simulink model "FMT_QuadPlantStep"  (R2026b)
settings: Solver=FixedStepDiscrete  StopTime=2  FixedStep=0.0005
undefined symbols (not defined in the file): PlantStepS
settings Model: DataDictionary=Flight_Parameters.sldd  Creator=26718  LastModifiedBy=26718

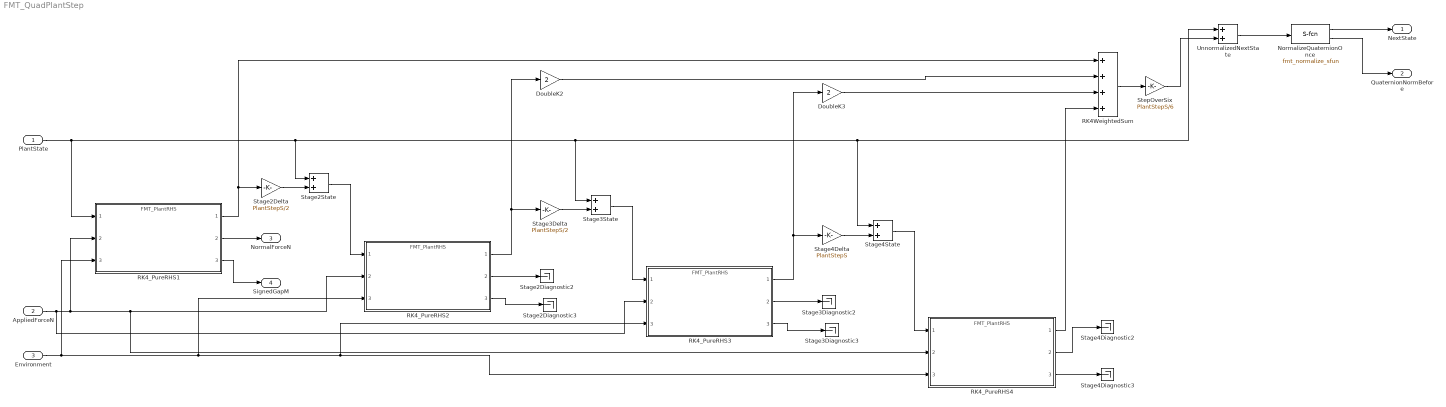
== system FMT_QuadPlantStep ==
  PlantState : Inport  OutDataTypeStr=double  PortDimensions=17
  AppliedForceN : Inport  Port=2  OutDataTypeStr=double  PortDimensions=4
  Environment : Inport  Port=3  OutDataTypeStr=double  PortDimensions=15
  DoubleK2 : Gain  Gain=2
  DoubleK3 : Gain  Gain=2
  NormalizeQuaternionOnce : S-Function  FunctionName=fmt_normalize_sfun  SFunctionDeploymentMode=off  EnableBusSupport=off
  RK4WeightedSum : Sum  Inputs=++++
  RK4_PureRHS{1..4} (4 alike) : ModelReference  ModelNameDialog=FMT_PlantRHS  SimulationMode=Normal  ModelReferenceVersion=1.1
  Stage2Delta : Gain  Gain=PlantStepS/2
  Stage2Diagnostic2 : Terminator
  Stage2Diagnostic3 : Terminator
  Stage2State : Sum
  Stage3Delta : Gain  Gain=PlantStepS/2
  Stage3Diagnostic2 : Terminator
  Stage3Diagnostic3 : Terminator
  Stage3State : Sum
  Stage4Delta : Gain  Gain=PlantStepS
  Stage4Diagnostic2 : Terminator
  Stage4Diagnostic3 : Terminator
  Stage4State : Sum
  StepOverSix : Gain  Gain=PlantStepS/6
  UnnormalizedNextState : Sum
  NextState : Outport
  QuaternionNormBefore : Outport  Port=2
  NormalForceN : Outport  Port=3
  SignedGapM : Outport  Port=4
  wires:
  NormalizeQuaternionOnce/2 -> QuaternionNormBefore/1
  NormalizeQuaternionOnce/1 -> NextState/1
  UnnormalizedNextState/1 -> NormalizeQuaternionOnce/1
  StepOverSix/1 -> UnnormalizedNextState/2
  RK4WeightedSum/1 -> StepOverSix/1
  RK4_PureRHS4/1 -> RK4WeightedSum/4
  DoubleK3/1 -> RK4WeightedSum/3
  DoubleK2/1 -> RK4WeightedSum/2
  RK4_PureRHS4/3 -> Stage4Diagnostic3/1
  RK4_PureRHS4/2 -> Stage4Diagnostic2/1
  Stage4State/1 -> RK4_PureRHS4/1
  Stage4Delta/1 -> Stage4State/2
  RK4_PureRHS3/1 -> Stage4Delta/1, DoubleK3/1
  RK4_PureRHS3/3 -> Stage3Diagnostic3/1
  RK4_PureRHS3/2 -> Stage3Diagnostic2/1
  Stage3State/1 -> RK4_PureRHS3/1
  Stage3Delta/1 -> Stage3State/2
  RK4_PureRHS2/1 -> Stage3Delta/1, DoubleK2/1
  RK4_PureRHS2/3 -> Stage2Diagnostic3/1
  RK4_PureRHS2/2 -> Stage2Diagnostic2/1
  Stage2State/1 -> RK4_PureRHS2/1
  Stage2Delta/1 -> Stage2State/2
  RK4_PureRHS1/1 -> Stage2Delta/1, RK4WeightedSum/1
  RK4_PureRHS1/3 -> SignedGapM/1
  RK4_PureRHS1/2 -> NormalForceN/1
  PlantState/1 -> UnnormalizedNextState/1, Stage4State/1, Stage3State/1, Stage2State/1, RK4_PureRHS1/1
  Environment/1 -> RK4_PureRHS3/3, RK4_PureRHS4/3, RK4_PureRHS2/3, RK4_PureRHS1/3
  AppliedForceN/1 -> RK4_PureRHS2/2, RK4_PureRHS4/2, RK4_PureRHS1/2, RK4_PureRHS3/2
